simulink model "sm_car"  (R2025a)
settings: Solver=ode23t  StartTime=0.0  StopTime=400  MaxStep=0.4  RelTol=1e-3  AbsTol=1e-3  EnableMultiTasking=on
PreLoadFcn:
  | % Due to usability issue in Repeating Sequence block
  | warning('off','Simulink:Masking:Invalid');
  | 
  | % Eliminate unnecessary warnings in inactive variants
  | % Warnings generated only if you click through inactive variant
  | warning('off','MATLAB:nonExistentField');
  | warning('off','Simulink:Parameters:BlkParamUndefined');
PostLoadFcn:
  | set_param([bdroot '/Vehicle'],'popup_trailer','Off')
  | warning('off','sm:sli:setup:compile:LocalSolverNotSupported')
  | %sm_car_config_maneuver(bdroot,'WOT Braking');
  | sm_car_config_vehicle(bdroot,'false');
  | sm_car_config_logging(bdroot);
InitFcn:
  | sm_car_config_camera;
  | Vehicle = sm_car_vehcfg_checkConfig(Vehicle);
  | sm_car_check_tire_model(bdroot);
StartFcn:
  | tic;
StopFcn:
  | Elapsed_Sim_Time = toc;
  | % disp(['Elapsed Sim Time = ' num2str(Elapsed_Sim_Time)]);
undefined symbols (not defined in the file): Axle1D, AxleIn, Camera, Control, Driver, Free, Init, Maneuver, Pedal, RaceFix, RaceSpin, Scene, ShaftL1, ShaftL2, ShaftR1, ShaftR2, Soft, Stiff, Visual, X, xy_data_car_side, Y, Z
libraries: sm_lib x1546, nesl_utility x528, fl_lib x480, SimscapeFluids_lib x61, sdl_lib x49, simulink x29, ee_lib x7, simulink_extras x6, Linkage_Systems x4, Tire_1x2x x4, AntiRollBar_Systems x2, Linkage_Decoupled x2
(part 57 of 79)

== system sm_car/Vehicle/Vehicle/Chassis/SuspA1/Linkage Decoupled/Steer/Rack Wheel/Driver/None ==
  q : Inport
  Body Sensor Empty : Subsystem  mask{offset_body_sensor=Vehicle.Chassis.Body.sCG.Value}
      mask prompts: offset_body_sensor "Sensor Frame Offset [x y z] (m)"
  Reference Frame : sm_lib/Frames and Transforms/Reference Frame
  Reference Frame1 : sm_lib/Frames and Transforms/Reference Frame
  Reference Frame2 : sm_lib/Frames and Transforms/Reference Frame
  Terminator : Terminator
  HandR : PMIOPort  Side=Right
  HandL : PMIOPort  Port=2  Side=Right
  Ref : PMIOPort  Port=3  Side=Left
  m : Outport  VectorParamsAs1DForOutWhenUnconnected=off
  wires:
  Body Sensor Empty/1(Body) -> m/1
  q/1 -> Terminator/1
  connections:
  Ref/RConn1 -- Reference Frame2/RConn1
  HandL/RConn1 -- Body Sensor Empty/LConn1 -- Reference Frame/RConn1
  Reference Frame1/RConn1 -- HandR/RConn1

== system sm_car/Vehicle/Vehicle/Chassis/SuspA1/Linkage Decoupled/Steer/Rack Wheel/Rack/Transform Suspension Mount ==
  Transform HP Rack : sm_lib/Frames and Transforms/Rigid Transform  RotationMethod=None  FollAlignAxisA=+X  BaseAlignAxisA=+Y  FollAlignAxisB=+Y  BaseAlignAxisB=+Z  RotationStandardAxis=+Z  RotationAngle=0.0  RotationAngleUnits=deg  RotationArbitraryAxis=[0 0 1]  RotationSequenceAxes=FollowerAxes  RotationSequence=XYX  RotationSequenceAngles=[0 0 0]  RotationSequenceAnglesUnits=deg  RotationMatrix=[1 0 0; 0 1 0; 0 0 1]  Quaternion=[1 0 0 0]  TranslationMethod=Cartesian  TranslationCartesianOffset=hp_mt_rack  TranslationCartesianOffsetUnits=m  TranslationStandardAxis=+Z  TranslationStandardOffset=0  TranslationStandardOffsetUnits=m  TranslationROffset=0  TranslationROffsetUnits=m  TranslationThetaOffset=0  TranslationThetaOffsetUnits=deg  TranslationZOffset=0  TranslationZOffsetUnits=m
  Transform Rack Axis : sm_lib/Frames and Transforms/Rigid Transform  RotationMethod=AlignedAxes  FollAlignAxisA=+Y  BaseAlignAxisA=-Z  FollAlignAxisB=+X  BaseAlignAxisB=+X  RotationStandardAxis=+Z  RotationAngle=0  RotationAngleUnits=deg  RotationArbitraryAxis=[0 0 1]  RotationSequenceAxes=FollowerAxes  RotationSequence=XYX  RotationSequenceAngles=[0 0 0]  RotationSequenceAnglesUnits=deg  RotationMatrix=[0 0 -1;0 1 0;1 0 0]  Quaternion=[1 0 0 0]  TranslationMethod=None  TranslationCartesianOffset=[0 0 0]  TranslationCartesianOffsetUnits=m  TranslationStandardAxis=+Z  TranslationStandardOffset=0  TranslationStandardOffsetUnits=m  TranslationROffset=0  TranslationROffsetUnits=m  TranslationThetaOffset=0  TranslationThetaOffsetUnits=deg  TranslationZOffset=0  TranslationZOffsetUnits=m
  B : PMIOPort  Side=Left
  F : PMIOPort  Port=2  Side=Right
  connections:
  Transform Rack Axis/LConn1 -- Transform HP Rack/RConn1
  Transform HP Rack/LConn1 -- B/RConn1
  Transform Rack Axis/RConn1 -- F/RConn1

== system sm_car/Vehicle/Vehicle/Chassis/SuspA1/Linkage Decoupled/Steer/Rack Wheel/Wheel/FSAE ==
  Solid : sm_lib/Body Elements/File Solid  ExtGeomFileName=FSAE_steering_wheel.STEP  UnitType=FromFile  ExtGeomFileUnits=m  StepReaderType=HEX  ExportConvexHullGeometry=off  InertiaType=PointMass  BasedOnType=Density  Density=1000  DensityUnits=kg/m^3  Mass=0  MassUnits=kg  CenterOfMass=[0 0 0]  CenterOfMassUnits=mm  MomentsOfInertia=[1 1 1]  MomentsOfInertiaUnits=kg*mm^2  ProductsOfInertia=[0 0 0]  ProductsOfInertiaUnits=kg*mm^2  GraphicType=FromGeometry  MarkerShape=Sphere  MarkerSize=10  GraphicVisPropType=SimpleVisualProperties  GraphicDiffuseColor=[0.898039215686275 0.917647058823529 0.929411764705882]  GraphicOpacity=1  GraphicSpecularColor=[0.5 0.5 0.5 1.0]  GraphicAmbientColor=[0.15 0.15 0.15 1.0]  GraphicEmissiveColor=[0.0 0.0 0.0 1.0]  GraphicShininess=75  DoExposeReferenceFrame=on  SerializedFrames=<Frames/>
  Transform HandL : sm_lib/Frames and Transforms/Rigid Transform  RotationMethod=AlignedAxes  FollAlignAxisA=+Z  BaseAlignAxisA=-Y  FollAlignAxisB=+X  BaseAlignAxisB=-Z  RotationStandardAxis=+Z  RotationAngle=0  RotationAngleUnits=rad  RotationArbitraryAxis=[0 0 0]  RotationSequenceAxes=FollowerAxes  RotationSequence=XYX  RotationSequenceAngles=[0 0 0]  RotationSequenceAnglesUnits=deg  RotationMatrix=[1 0 0; 0 1 0; 0 0 1]  Quaternion=[1 0 0 0]  TranslationMethod=Cartesian  TranslationCartesianOffset=[-20 130 -10]  TranslationCartesianOffsetUnits=mm  TranslationStandardAxis=+Z  TranslationStandardOffset=0  TranslationStandardOffsetUnits=mm  TranslationROffset=0  TranslationROffsetUnits=m  TranslationThetaOffset=0  TranslationThetaOffsetUnits=deg  TranslationZOffset=0  TranslationZOffsetUnits=m
  Transform HandL Pitch : sm_lib/Frames and Transforms/Rigid Transform  RotationMethod=StandardAxis  FollAlignAxisA=+X  BaseAlignAxisA=+Y  FollAlignAxisB=+Y  BaseAlignAxisB=+Z  RotationStandardAxis=+Z  RotationAngle=20  RotationAngleUnits=deg  RotationArbitraryAxis=[0 0 1]  RotationSequenceAxes=FollowerAxes  RotationSequence=XYX  RotationSequenceAngles=[0 0 0]  RotationSequenceAnglesUnits=deg  RotationMatrix=[1 0 0; 0 1 0; 0 0 1]  Quaternion=[1 0 0 0]  TranslationMethod=None  TranslationCartesianOffset=[0 0 0]  TranslationCartesianOffsetUnits=m  TranslationStandardAxis=+Z  TranslationStandardOffset=0  TranslationStandardOffsetUnits=m  TranslationROffset=0  TranslationROffsetUnits=m  TranslationThetaOffset=0  TranslationThetaOffsetUnits=deg  TranslationZOffset=0  TranslationZOffsetUnits=m
  Transform HandR : sm_lib/Frames and Transforms/Rigid Transform  RotationMethod=AlignedAxes  FollAlignAxisA=+Z  BaseAlignAxisA=-Y  FollAlignAxisB=+X  BaseAlignAxisB=-Z  RotationStandardAxis=+Z  RotationAngle=0  RotationAngleUnits=rad  RotationArbitraryAxis=[0 0 0]  RotationSequenceAxes=FollowerAxes  RotationSequence=XYX  RotationSequenceAngles=[0 0 0]  RotationSequenceAnglesUnits=deg  RotationMatrix=[1 0 0; 0 1 0; 0 0 1]  Quaternion=[1 0 0 0]  TranslationMethod=Cartesian  TranslationCartesianOffset=[-20 -130 -10]  TranslationCartesianOffsetUnits=mm  TranslationStandardAxis=+Z  TranslationStandardOffset=0  TranslationStandardOffsetUnits=mm  TranslationROffset=0  TranslationROffsetUnits=m  TranslationThetaOffset=0  TranslationThetaOffsetUnits=deg  TranslationZOffset=0  TranslationZOffsetUnits=m
  Transform HandR Pitch : sm_lib/Frames and Transforms/Rigid Transform  RotationMethod=StandardAxis  FollAlignAxisA=+X  BaseAlignAxisA=+Y  FollAlignAxisB=+Y  BaseAlignAxisB=+Z  RotationStandardAxis=+Z  RotationAngle=20  RotationAngleUnits=deg  RotationArbitraryAxis=[0 0 1]  RotationSequenceAxes=FollowerAxes  RotationSequence=XYX  RotationSequenceAngles=[0 0 0]  RotationSequenceAnglesUnits=deg  RotationMatrix=[1 0 0; 0 1 0; 0 0 1]  Quaternion=[1 0 0 0]  TranslationMethod=None  TranslationCartesianOffset=[0 0 0]  TranslationCartesianOffsetUnits=m  TranslationStandardAxis=+Z  TranslationStandardOffset=0  TranslationStandardOffsetUnits=m  TranslationROffset=0  TranslationROffsetUnits=m  TranslationThetaOffset=0  TranslationThetaOffsetUnits=deg  TranslationZOffset=0  TranslationZOffsetUnits=m
  Transform Steer Axis : Subsystem
  "SteerAxis  " : PMIOPort  Side=Left
  HandR : PMIOPort  Port=2  Side=Right
  HandL : PMIOPort  Port=3  Side=Right
  connections:
  Transform HandR Pitch/RConn1 -- HandR/RConn1
  Transform HandL Pitch/LConn1 -- Transform HandL/RConn1
  Solid/RConn1 -- Transform Steer Axis/RConn1
  HandL/RConn1 -- Transform HandL Pitch/RConn1
  Transform HandR/RConn1 -- Transform HandR Pitch/LConn1
  Transform Steer Axis/LConn1 -- Transform HandL/LConn1 -- Transform HandR/LConn1 -- "SteerAxis  "/RConn1

== system sm_car/Vehicle/Vehicle/Chassis/SuspA1/Linkage Decoupled/Steer/Rack Wheel/Wheel/Sedan ==
  Reference Frame : sm_lib/Frames and Transforms/Reference Frame
  Steering : Subsystem
  Transform Align HandL : sm_lib/Frames and Transforms/Rigid Transform  RotationMethod=None  FollAlignAxisA=+X  BaseAlignAxisA=+Y  FollAlignAxisB=+Y  BaseAlignAxisB=+Z  RotationStandardAxis=+Z  RotationAngle=0  RotationAngleUnits=deg  RotationArbitraryAxis=[0 0 1]  RotationSequenceAxes=FollowerAxes  RotationSequence=XYX  RotationSequenceAngles=[0 0 0]  RotationSequenceAnglesUnits=deg  RotationMatrix=[1 0 0; 0 1 0; 0 0 1]  Quaternion=[1 0 0 0]  TranslationMethod=StandardAxis  TranslationCartesianOffset=[0 0 0]  TranslationCartesianOffsetUnits=m  TranslationStandardAxis=+Z  TranslationStandardOffset=0.01  TranslationStandardOffsetUnits=m  TranslationROffset=0  TranslationROffsetUnits=m  TranslationThetaOffset=0  TranslationThetaOffsetUnits=deg  TranslationZOffset=0  TranslationZOffsetUnits=m
  Transform HandL : sm_lib/Frames and Transforms/Rigid Transform  RotationMethod=ArbitraryAxis  FollAlignAxisA=+X  BaseAlignAxisA=+Y  FollAlignAxisB=+Y  BaseAlignAxisB=+Z  RotationStandardAxis=+Z  RotationAngle=0  RotationAngleUnits=rad  RotationArbitraryAxis=[0 0 0]  RotationSequenceAxes=FollowerAxes  RotationSequence=XYX  RotationSequenceAngles=[0 0 0]  RotationSequenceAnglesUnits=deg  RotationMatrix=[1 0 0; 0 1 0; 0 0 1]  Quaternion=[1 0 0 0]  TranslationMethod=Cartesian  TranslationCartesianOffset=[75.3002166748051 139.529690146446 17.4556095153098]  TranslationCartesianOffsetUnits=mm  TranslationStandardAxis=+Z  TranslationStandardOffset=0  TranslationStandardOffsetUnits=mm  TranslationROffset=0  TranslationROffsetUnits=m  TranslationThetaOffset=0  TranslationThetaOffsetUnits=deg  TranslationZOffset=0  TranslationZOffsetUnits=m
  Transform Steer Ctr : sm_lib/Frames and Transforms/Rigid Transform  RotationMethod=RotationSequence  FollAlignAxisA=+X  BaseAlignAxisA=+Y  FollAlignAxisB=+Y  BaseAlignAxisB=+Z  RotationStandardAxis=+Z  RotationAngle=0  RotationAngleUnits=deg  RotationArbitraryAxis=[0 0 1]  RotationSequenceAxes=FollowerAxes  RotationSequence=YXZ  RotationSequenceAngles=[-90 -20.218116663649042 90]  RotationSequenceAnglesUnits=deg  RotationMatrix=[1 0 0; 0 1 0; 0 0 1]  Quaternion=[1 0 0 0]  TranslationMethod=Cartesian  TranslationCartesianOffset=[0.072679731994867 0.197345148772001 0]  TranslationCartesianOffsetUnits=m  TranslationStandardAxis=+Z  TranslationStandardOffset=0  TranslationStandardOffsetUnits=m  TranslationROffset=0  TranslationROffsetUnits=m  TranslationThetaOffset=0  TranslationThetaOffsetUnits=deg  TranslationZOffset=0  TranslationZOffsetUnits=m
  Transform HandR : sm_lib/Frames and Transforms/Rigid Transform  RotationMethod=ArbitraryAxis  FollAlignAxisA=+X  BaseAlignAxisA=+Y  FollAlignAxisB=+Y  BaseAlignAxisB=+Z  RotationStandardAxis=+Z  RotationAngle=0  RotationAngleUnits=rad  RotationArbitraryAxis=[0 0 0]  RotationSequenceAxes=FollowerAxes  RotationSequence=XYX  RotationSequenceAngles=[0 0 0]  RotationSequenceAnglesUnits=deg  RotationMatrix=[1 0 0; 0 1 0; 0 0 1]  Quaternion=[1 0 0 0]  TranslationMethod=Cartesian  TranslationCartesianOffset=[75.3002166748047 139.529690146446 404.207736253739]  TranslationCartesianOffsetUnits=mm  TranslationStandardAxis=+Z  TranslationStandardOffset=0  TranslationStandardOffsetUnits=mm  TranslationROffset=0  TranslationROffsetUnits=m  TranslationThetaOffset=0  TranslationThetaOffsetUnits=deg  TranslationZOffset=0  TranslationZOffsetUnits=m
  SteerAxis : PMIOPort  Side=Left
  HandR : PMIOPort  Port=2  Side=Right
  HandL : PMIOPort  Port=3  Side=Right
  connections:
  SteerAxis/RConn1 -- Transform Steer Ctr/RConn1
  Transform HandL/RConn1 -- Transform Align HandL/LConn1
  Steering/LConn1 -- Transform Steer Ctr/LConn1
  Transform Align HandL/RConn1 -- HandL/RConn1
  Transform HandR/RConn1 -- HandR/RConn1
  Transform HandR/LConn1 -- Steering/RConn1 -- Transform HandL/LConn1
  Steering/LConn2 -- Reference Frame/RConn1

== system sm_car/Vehicle/Vehicle/Chassis/SuspA1/Linkage Decoupled/Steer/Rack Wheel ByWire/Driver/Human ==
  q : Inport
  Arm L : Subsystem
  Arm R : Subsystem
  Body Sensor : Subsystem  mask{offset_body_sensor=Vehicle.Chassis.Body.sCG.Value}
      mask prompts: offset_body_sensor "Sensor Frame Offset [x y z] (m)"
  Gain : Gain  Gain=-1
  Head : Subsystem
  Leg L : Subsystem
  Leg R : Subsystem
  Pelvis : Subsystem
  Revolute Neck : sm_lib/Joints/Revolute Joint  JointMode=Normal  CompositeWrenchDir=FollowerOnBase  CompositeWrenchFrame=BaseFrame  SenseConstraintForce=off  SenseConstraintTorque=off  SenseTotalForce=off  SenseTotalTorque=off  PositionTargetSpecify=on  PositionTargetPriority=Low  PositionTargetValue=0  PositionTargetValueUnits=deg  VelocityTargetSpecify=off  VelocityTargetPriority=High  VelocityTargetValue=0  VelocityTargetValueUnits=deg/s  EquilibriumPosition=0  EquilibriumPositionUnits=rad  SpringStiffness=0  SpringStiffnessUnits=N*m/rad  DampingCoefficient=0  DampingCoefficientUnits=N*m/(rad/s)  LowerLimitSpecify=off  LowerLimitBound=-90  LowerLimitBoundUnits=deg  LowerLimitStiffness=1e4  LowerLimitStiffnessUnits=N*m/deg  LowerLimitDamping=10  LowerLimitDampingUnits=N*m/(deg/s)  LowerLimitTransitionRegionWidth=0.1  LowerLimitTransitionRegionWidthUnits=deg  UpperLimitSpecify=off  UpperLimitBound=90  UpperLimitBoundUnits=deg  UpperLimitStiffness=1e4  UpperLimitStiffnessUnits=N*m/deg  UpperLimitDamping=10  UpperLimitDampingUnits=N*m/(deg/s)  UpperLimitTransitionRegionWidth=0.1  UpperLimitTransitionRegionWidthUnits=deg  TorqueActuationMode=ComputedTorque  MotionActuationMode=InputMotion  SensePosition=off  SenseVelocity=off  SenseAcceleration=off  SenseTorqueForce=off  SenseLowerLimitTorqueForce=off  SenseUpperLimitTorqueForce=off
  Simulink-PS Converter : nesl_utility/Simulink-PS Converter  PhysicalDomain=network_engine_domain  SubClassName=ps_input  LeftPortType=input  RightPortType=output  PseudoPeriodic=off  Frequencies=[]  NoiseDistribution=none  NoiseParameters=[]  Unit=rad  AffineConversion=off  FilteringAndDerivatives=filter  SimscapeFilterOrder=2  InputFilterTimeConstant=0.1  UdotUserProvided=0
  Torso : Subsystem
  Transform FA to Driver : sm_lib/Frames and Transforms/Rigid Transform  RotationMethod=RotationSequence  FollAlignAxisA=+X  BaseAlignAxisA=+Y  FollAlignAxisB=+Y  BaseAlignAxisB=+Z  RotationStandardAxis=+Z  RotationAngle=0.0  RotationAngleUnits=deg  RotationArbitraryAxis=[0 0 1]  RotationSequenceAxes=FollowerAxes  RotationSequence=ZYX  RotationSequenceAngles=[rpy_human(3) rpy_human(2) rpy_human(1)]  RotationSequenceAnglesUnits=deg  RotationMatrix=[1 0 0; 0 1 0; 0 0 1]  Quaternion=[1 0 0 0]  TranslationMethod=Cartesian  TranslationCartesianOffset=hp_human  TranslationCartesianOffsetUnits=m  TranslationStandardAxis=+Z  TranslationStandardOffset=0  TranslationStandardOffsetUnits=m  TranslationROffset=0  TranslationROffsetUnits=m  TranslationThetaOffset=0  TranslationThetaOffsetUnits=deg  TranslationZOffset=0  TranslationZOffsetUnits=m
  Transform Seat Angle : sm_lib/Frames and Transforms/Rigid Transform  RotationMethod=StandardAxis  FollAlignAxisA=+X  BaseAlignAxisA=+Y  FollAlignAxisB=+Y  BaseAlignAxisB=+Z  RotationStandardAxis=+Y  RotationAngle=143.2261743756  RotationAngleUnits=deg  RotationArbitraryAxis=[0 0 1]  RotationSequenceAxes=FollowerAxes  RotationSequence=XYX  RotationSequenceAngles=[0 0 0]  RotationSequenceAnglesUnits=deg  RotationMatrix=[1 0 0; 0 1 0; 0 0 1]  Quaternion=[1 0 0 0]  TranslationMethod=None  TranslationCartesianOffset=[0 0 0]  TranslationCartesianOffsetUnits=m  TranslationStandardAxis=+Z  TranslationStandardOffset=0  TranslationStandardOffsetUnits=m  TranslationROffset=0  TranslationROffsetUnits=m  TranslationThetaOffset=0  TranslationThetaOffsetUnits=deg  TranslationZOffset=0  TranslationZOffsetUnits=m
  Twist : Subsystem
  HandR : PMIOPort  Side=Right
  HandL : PMIOPort  Port=2  Side=Right
  Ref : PMIOPort  Port=3  Side=Left
  m : Outport  VectorParamsAs1DForOutWhenUnconnected=off
  wires:
  Body Sensor/1(Body) -> m/1
  Gain/1 -> Simulink-PS Converter/1
  q/1 -> Gain/1
  connections:
  Body Sensor/LConn1 -- Head/RConn1
  Transform Seat Angle/RConn1 -- Transform FA to Driver/RConn1
  Head/LConn1 -- Revolute Neck/RConn1
  Revolute Neck/LConn1 -- Torso/RConn2
  Pelvis/RConn2 -- Leg R/LConn1
  Leg L/LConn1 -- Pelvis/RConn1
  Arm R/RConn1 -- HandR/RConn1
  Torso/RConn3 -- Arm R/LConn1
  Arm L/LConn1 -- Torso/RConn1
  Arm L/RConn1 -- HandL/RConn1
  Twist/RConn1 -- Torso/LConn1
  Pelvis/LConn1 -- Twist/LConn1 -- Transform Seat Angle/LConn1
  Transform FA to Driver/LConn1 -- Ref/RConn1
  Simulink-PS Converter/RConn1 -- Revolute Neck/LConn2

== system sm_car/Vehicle/Vehicle/Chassis/SuspA1/Linkage Decoupled/Steer/Rack Wheel ByWire/Driver/None ==
  q : Inport
  Body Sensor Empty : Subsystem  mask{offset_body_sensor=Vehicle.Chassis.Body.sCG.Value}
      mask prompts: offset_body_sensor "Sensor Frame Offset [x y z] (m)"
  Reference Frame : sm_lib/Frames and Transforms/Reference Frame
  Reference Frame1 : sm_lib/Frames and Transforms/Reference Frame
  Reference Frame2 : sm_lib/Frames and Transforms/Reference Frame
  Terminator : Terminator
  HandR : PMIOPort  Side=Right
  HandL : PMIOPort  Port=2  Side=Right
  Ref : PMIOPort  Port=3  Side=Left
  m : Outport  VectorParamsAs1DForOutWhenUnconnected=off
  wires:
  Body Sensor Empty/1(Body) -> m/1
  q/1 -> Terminator/1
  connections:
  Ref/RConn1 -- Reference Frame2/RConn1
  HandL/RConn1 -- Body Sensor Empty/LConn1 -- Reference Frame/RConn1
  Reference Frame1/RConn1 -- HandR/RConn1

== system sm_car/Vehicle/Vehicle/Chassis/SuspA1/Linkage Decoupled/Steer/Rack Wheel ByWire/Motors/Control ==
  Meas : Inport
  Cmd : Inport  Port=2
  Abs : Abs  ZeroCross=off  SaturateOnIntegerOverflow=off
  Derivative : TransferFcn  Numerator=[1 0]  Denominator=[tFilt_deriv 1]
  Filter xRack : simulink_extras/Additional Linear/Transfer Fcn (with initial states)  N=[1]  D=[tFilt_xRack 1]  X0=0
  Integrator : Integrator
  Kd : Gain  Gain=Kd
  Ki : Gain  Gain=Ki
  Kp : Lookup_n-D  NumberOfTableDimensions=1  BreakpointsForDimension1=Kp_breakpoints  Table=Kp_values  InternalRulePriority=Speed  RndMeth=Simplest
  Product : Product
  Product1 : Product
  Steer Torque Factor : Constant  Value=nTrqSteer
  Sum : Sum  Inputs=+-|
  Sum1 : Sum  Inputs=+++
  trqRack : Outport
  trqSteer : Outport  Port=2
  wires:
  Cmd/1 -> Sum/1, Abs/1
  Meas/1 -> Filter xRack/1
  Sum/1 -> Ki/1, Product/2, Kd/1
  Integrator/1 -> Sum1/2
  Ki/1 -> Integrator/1
  Product/1 -> Sum1/1
  Kd/1 -> Derivative/1
  Derivative/1 -> Sum1/3
  Filter xRack/1 -> Sum/2
  Kp/1 -> Product/1
  Abs/1 -> Kp/1
  Steer Torque Factor/1 -> Product1/1
  Product1/1 -> trqSteer/1
  Sum1/1 -> Product1/2, trqRack/1

== system sm_car/Vehicle/Vehicle/Chassis/SuspA1/Linkage Decoupled/Steer/Rack Wheel ByWire/Rack/Transform Suspension Mount ==
  Transform HP Rack : sm_lib/Frames and Transforms/Rigid Transform  RotationMethod=None  FollAlignAxisA=+X  BaseAlignAxisA=+Y  FollAlignAxisB=+Y  BaseAlignAxisB=+Z  RotationStandardAxis=+Z  RotationAngle=0.0  RotationAngleUnits=deg  RotationArbitraryAxis=[0 0 1]  RotationSequenceAxes=FollowerAxes  RotationSequence=XYX  RotationSequenceAngles=[0 0 0]  RotationSequenceAnglesUnits=deg  RotationMatrix=[1 0 0; 0 1 0; 0 0 1]  Quaternion=[1 0 0 0]  TranslationMethod=Cartesian  TranslationCartesianOffset=hp_mt_rack  TranslationCartesianOffsetUnits=m  TranslationStandardAxis=+Z  TranslationStandardOffset=0  TranslationStandardOffsetUnits=m  TranslationROffset=0  TranslationROffsetUnits=m  TranslationThetaOffset=0  TranslationThetaOffsetUnits=deg  TranslationZOffset=0  TranslationZOffsetUnits=m
  Transform Rack Axis : sm_lib/Frames and Transforms/Rigid Transform  RotationMethod=AlignedAxes  FollAlignAxisA=+Y  BaseAlignAxisA=-Z  FollAlignAxisB=+X  BaseAlignAxisB=+X  RotationStandardAxis=+Z  RotationAngle=0  RotationAngleUnits=deg  RotationArbitraryAxis=[0 0 1]  RotationSequenceAxes=FollowerAxes  RotationSequence=XYX  RotationSequenceAngles=[0 0 0]  RotationSequenceAnglesUnits=deg  RotationMatrix=[0 0 -1;0 1 0;1 0 0]  Quaternion=[1 0 0 0]  TranslationMethod=None  TranslationCartesianOffset=[0 0 0]  TranslationCartesianOffsetUnits=m  TranslationStandardAxis=+Z  TranslationStandardOffset=0  TranslationStandardOffsetUnits=m  TranslationROffset=0  TranslationROffsetUnits=m  TranslationThetaOffset=0  TranslationThetaOffsetUnits=deg  TranslationZOffset=0  TranslationZOffsetUnits=m
  B : PMIOPort  Side=Left
  F : PMIOPort  Port=2  Side=Right
  connections:
  Transform Rack Axis/LConn1 -- Transform HP Rack/RConn1
  Transform HP Rack/LConn1 -- B/RConn1
  Transform Rack Axis/RConn1 -- F/RConn1

== system sm_car/Vehicle/Vehicle/Chassis/SuspA1/Linkage Decoupled/Steer/Rack Wheel ByWire/Wheel/FSAE ==
  Solid : sm_lib/Body Elements/File Solid  ExtGeomFileName=FSAE_steering_wheel.STEP  UnitType=FromFile  ExtGeomFileUnits=m  StepReaderType=HEX  ExportConvexHullGeometry=off  InertiaType=PointMass  BasedOnType=Density  Density=1000  DensityUnits=kg/m^3  Mass=0  MassUnits=kg  CenterOfMass=[0 0 0]  CenterOfMassUnits=mm  MomentsOfInertia=[1 1 1]  MomentsOfInertiaUnits=kg*mm^2  ProductsOfInertia=[0 0 0]  ProductsOfInertiaUnits=kg*mm^2  GraphicType=FromGeometry  MarkerShape=Sphere  MarkerSize=10  GraphicVisPropType=SimpleVisualProperties  GraphicDiffuseColor=[0.898039215686275 0.917647058823529 0.929411764705882]  GraphicOpacity=1  GraphicSpecularColor=[0.5 0.5 0.5 1.0]  GraphicAmbientColor=[0.15 0.15 0.15 1.0]  GraphicEmissiveColor=[0.0 0.0 0.0 1.0]  GraphicShininess=75  DoExposeReferenceFrame=on  SerializedFrames=<Frames/>
  Transform HandL : sm_lib/Frames and Transforms/Rigid Transform  RotationMethod=AlignedAxes  FollAlignAxisA=+Z  BaseAlignAxisA=-Y  FollAlignAxisB=+X  BaseAlignAxisB=-Z  RotationStandardAxis=+Z  RotationAngle=0  RotationAngleUnits=rad  RotationArbitraryAxis=[0 0 0]  RotationSequenceAxes=FollowerAxes  RotationSequence=XYX  RotationSequenceAngles=[0 0 0]  RotationSequenceAnglesUnits=deg  RotationMatrix=[1 0 0; 0 1 0; 0 0 1]  Quaternion=[1 0 0 0]  TranslationMethod=Cartesian  TranslationCartesianOffset=[-20 130 -10]  TranslationCartesianOffsetUnits=mm  TranslationStandardAxis=+Z  TranslationStandardOffset=0  TranslationStandardOffsetUnits=mm  TranslationROffset=0  TranslationROffsetUnits=m  TranslationThetaOffset=0  TranslationThetaOffsetUnits=deg  TranslationZOffset=0  TranslationZOffsetUnits=m
  Transform HandL Pitch : sm_lib/Frames and Transforms/Rigid Transform  RotationMethod=StandardAxis  FollAlignAxisA=+X  BaseAlignAxisA=+Y  FollAlignAxisB=+Y  BaseAlignAxisB=+Z  RotationStandardAxis=+Z  RotationAngle=20  RotationAngleUnits=deg  RotationArbitraryAxis=[0 0 1]  RotationSequenceAxes=FollowerAxes  RotationSequence=XYX  RotationSequenceAngles=[0 0 0]  RotationSequenceAnglesUnits=deg  RotationMatrix=[1 0 0; 0 1 0; 0 0 1]  Quaternion=[1 0 0 0]  TranslationMethod=None  TranslationCartesianOffset=[0 0 0]  TranslationCartesianOffsetUnits=m  TranslationStandardAxis=+Z  TranslationStandardOffset=0  TranslationStandardOffsetUnits=m  TranslationROffset=0  TranslationROffsetUnits=m  TranslationThetaOffset=0  TranslationThetaOffsetUnits=deg  TranslationZOffset=0  TranslationZOffsetUnits=m
  Transform HandR : sm_lib/Frames and Transforms/Rigid Transform  RotationMethod=AlignedAxes  FollAlignAxisA=+Z  BaseAlignAxisA=-Y  FollAlignAxisB=+X  BaseAlignAxisB=-Z  RotationStandardAxis=+Z  RotationAngle=0  RotationAngleUnits=rad  RotationArbitraryAxis=[0 0 0]  RotationSequenceAxes=FollowerAxes  RotationSequence=XYX  RotationSequenceAngles=[0 0 0]  RotationSequenceAnglesUnits=deg  RotationMatrix=[1 0 0; 0 1 0; 0 0 1]  Quaternion=[1 0 0 0]  TranslationMethod=Cartesian  TranslationCartesianOffset=[-20 -130 -10]  TranslationCartesianOffsetUnits=mm  TranslationStandardAxis=+Z  TranslationStandardOffset=0  TranslationStandardOffsetUnits=mm  TranslationROffset=0  TranslationROffsetUnits=m  TranslationThetaOffset=0  TranslationThetaOffsetUnits=deg  TranslationZOffset=0  TranslationZOffsetUnits=m
  Transform HandR Pitch : sm_lib/Frames and Transforms/Rigid Transform  RotationMethod=StandardAxis  FollAlignAxisA=+X  BaseAlignAxisA=+Y  FollAlignAxisB=+Y  BaseAlignAxisB=+Z  RotationStandardAxis=+Z  RotationAngle=20  RotationAngleUnits=deg  RotationArbitraryAxis=[0 0 1]  RotationSequenceAxes=FollowerAxes  RotationSequence=XYX  RotationSequenceAngles=[0 0 0]  RotationSequenceAnglesUnits=deg  RotationMatrix=[1 0 0; 0 1 0; 0 0 1]  Quaternion=[1 0 0 0]  TranslationMethod=None  TranslationCartesianOffset=[0 0 0]  TranslationCartesianOffsetUnits=m  TranslationStandardAxis=+Z  TranslationStandardOffset=0  TranslationStandardOffsetUnits=m  TranslationROffset=0  TranslationROffsetUnits=m  TranslationThetaOffset=0  TranslationThetaOffsetUnits=deg  TranslationZOffset=0  TranslationZOffsetUnits=m
  Transform Steer Axis : Subsystem
  "SteerAxis  " : PMIOPort  Side=Left
  HandR : PMIOPort  Port=2  Side=Right
  HandL : PMIOPort  Port=3  Side=Right
  connections:
  Transform HandR Pitch/RConn1 -- HandR/RConn1
  Transform HandL Pitch/LConn1 -- Transform HandL/RConn1
  Solid/RConn1 -- Transform Steer Axis/RConn1
  HandL/RConn1 -- Transform HandL Pitch/RConn1
  Transform HandR/RConn1 -- Transform HandR Pitch/LConn1
  Transform Steer Axis/LConn1 -- Transform HandL/LConn1 -- Transform HandR/LConn1 -- "SteerAxis  "/RConn1

== system sm_car/Vehicle/Vehicle/Chassis/SuspA1/Linkage Decoupled/Steer/Rack Wheel ByWire/Wheel/Sedan ==
  Reference Frame : sm_lib/Frames and Transforms/Reference Frame
  Steering : Subsystem
  Transform Align HandL : sm_lib/Frames and Transforms/Rigid Transform  RotationMethod=None  FollAlignAxisA=+X  BaseAlignAxisA=+Y  FollAlignAxisB=+Y  BaseAlignAxisB=+Z  RotationStandardAxis=+Z  RotationAngle=0  RotationAngleUnits=deg  RotationArbitraryAxis=[0 0 1]  RotationSequenceAxes=FollowerAxes  RotationSequence=XYX  RotationSequenceAngles=[0 0 0]  RotationSequenceAnglesUnits=deg  RotationMatrix=[1 0 0; 0 1 0; 0 0 1]  Quaternion=[1 0 0 0]  TranslationMethod=StandardAxis  TranslationCartesianOffset=[0 0 0]  TranslationCartesianOffsetUnits=m  TranslationStandardAxis=+Z  TranslationStandardOffset=0.01  TranslationStandardOffsetUnits=m  TranslationROffset=0  TranslationROffsetUnits=m  TranslationThetaOffset=0  TranslationThetaOffsetUnits=deg  TranslationZOffset=0  TranslationZOffsetUnits=m
  Transform HandL : sm_lib/Frames and Transforms/Rigid Transform  RotationMethod=ArbitraryAxis  FollAlignAxisA=+X  BaseAlignAxisA=+Y  FollAlignAxisB=+Y  BaseAlignAxisB=+Z  RotationStandardAxis=+Z  RotationAngle=0  RotationAngleUnits=rad  RotationArbitraryAxis=[0 0 0]  RotationSequenceAxes=FollowerAxes  RotationSequence=XYX  RotationSequenceAngles=[0 0 0]  RotationSequenceAnglesUnits=deg  RotationMatrix=[1 0 0; 0 1 0; 0 0 1]  Quaternion=[1 0 0 0]  TranslationMethod=Cartesian  TranslationCartesianOffset=[75.3002166748051 139.529690146446 17.4556095153098]  TranslationCartesianOffsetUnits=mm  TranslationStandardAxis=+Z  TranslationStandardOffset=0  TranslationStandardOffsetUnits=mm  TranslationROffset=0  TranslationROffsetUnits=m  TranslationThetaOffset=0  TranslationThetaOffsetUnits=deg  TranslationZOffset=0  TranslationZOffsetUnits=m
  Transform Steer Ctr : sm_lib/Frames and Transforms/Rigid Transform  RotationMethod=RotationSequence  FollAlignAxisA=+X  BaseAlignAxisA=+Y  FollAlignAxisB=+Y  BaseAlignAxisB=+Z  RotationStandardAxis=+Z  RotationAngle=0  RotationAngleUnits=deg  RotationArbitraryAxis=[0 0 1]  RotationSequenceAxes=FollowerAxes  RotationSequence=YXZ  RotationSequenceAngles=[-90 -20.218116663649042 90]  RotationSequenceAnglesUnits=deg  RotationMatrix=[1 0 0; 0 1 0; 0 0 1]  Quaternion=[1 0 0 0]  TranslationMethod=Cartesian  TranslationCartesianOffset=[0.072679731994867 0.197345148772001 0]  TranslationCartesianOffsetUnits=m  TranslationStandardAxis=+Z  TranslationStandardOffset=0  TranslationStandardOffsetUnits=m  TranslationROffset=0  TranslationROffsetUnits=m  TranslationThetaOffset=0  TranslationThetaOffsetUnits=deg  TranslationZOffset=0  TranslationZOffsetUnits=m
  Transform HandR : sm_lib/Frames and Transforms/Rigid Transform  RotationMethod=ArbitraryAxis  FollAlignAxisA=+X  BaseAlignAxisA=+Y  FollAlignAxisB=+Y  BaseAlignAxisB=+Z  RotationStandardAxis=+Z  RotationAngle=0  RotationAngleUnits=rad  RotationArbitraryAxis=[0 0 0]  RotationSequenceAxes=FollowerAxes  RotationSequence=XYX  RotationSequenceAngles=[0 0 0]  RotationSequenceAnglesUnits=deg  RotationMatrix=[1 0 0; 0 1 0; 0 0 1]  Quaternion=[1 0 0 0]  TranslationMethod=Cartesian  TranslationCartesianOffset=[75.3002166748047 139.529690146446 404.207736253739]  TranslationCartesianOffsetUnits=mm  TranslationStandardAxis=+Z  TranslationStandardOffset=0  TranslationStandardOffsetUnits=mm  TranslationROffset=0  TranslationROffsetUnits=m  TranslationThetaOffset=0  TranslationThetaOffsetUnits=deg  TranslationZOffset=0  TranslationZOffsetUnits=m
  SteerAxis : PMIOPort  Side=Left
  HandR : PMIOPort  Port=2  Side=Right
  HandL : PMIOPort  Port=3  Side=Right
  connections:
  SteerAxis/RConn1 -- Transform Steer Ctr/RConn1
  Transform HandL/RConn1 -- Transform Align HandL/LConn1
  Steering/LConn1 -- Transform Steer Ctr/LConn1
  Transform Align HandL/RConn1 -- HandL/RConn1
  Transform HandR/RConn1 -- HandR/RConn1
  Transform HandR/LConn1 -- Steering/RConn1 -- Transform HandL/LConn1
  Steering/LConn2 -- Reference Frame/RConn1

== system sm_car/Vehicle/Vehicle/Chassis/SuspA1/Linkage Decoupled/Steer/Rack Wheel Indep/Driver/Human ==
  q : Inport
  Arm L : Subsystem
  Arm R : Subsystem
  Body Sensor : Subsystem  mask{offset_body_sensor=Vehicle.Chassis.Body.sCG.Value}
      mask prompts: offset_body_sensor "Sensor Frame Offset [x y z] (m)"
  Gain : Gain  Gain=-1
  Head : Subsystem
  Leg L : Subsystem
  Leg R : Subsystem
  Pelvis : Subsystem
  Revolute Neck : sm_lib/Joints/Revolute Joint  JointMode=Normal  CompositeWrenchDir=FollowerOnBase  CompositeWrenchFrame=BaseFrame  SenseConstraintForce=off  SenseConstraintTorque=off  SenseTotalForce=off  SenseTotalTorque=off  PositionTargetSpecify=on  PositionTargetPriority=Low  PositionTargetValue=0  PositionTargetValueUnits=deg  VelocityTargetSpecify=off  VelocityTargetPriority=High  VelocityTargetValue=0  VelocityTargetValueUnits=deg/s  EquilibriumPosition=0  EquilibriumPositionUnits=rad  SpringStiffness=0  SpringStiffnessUnits=N*m/rad  DampingCoefficient=0  DampingCoefficientUnits=N*m/(rad/s)  LowerLimitSpecify=off  LowerLimitBound=-90  LowerLimitBoundUnits=deg  LowerLimitStiffness=1e4  LowerLimitStiffnessUnits=N*m/deg  LowerLimitDamping=10  LowerLimitDampingUnits=N*m/(deg/s)  LowerLimitTransitionRegionWidth=0.1  LowerLimitTransitionRegionWidthUnits=deg  UpperLimitSpecify=off  UpperLimitBound=90  UpperLimitBoundUnits=deg  UpperLimitStiffness=1e4  UpperLimitStiffnessUnits=N*m/deg  UpperLimitDamping=10  UpperLimitDampingUnits=N*m/(deg/s)  UpperLimitTransitionRegionWidth=0.1  UpperLimitTransitionRegionWidthUnits=deg  TorqueActuationMode=ComputedTorque  MotionActuationMode=InputMotion  SensePosition=off  SenseVelocity=off  SenseAcceleration=off  SenseTorqueForce=off  SenseLowerLimitTorqueForce=off  SenseUpperLimitTorqueForce=off
  Simulink-PS Converter : nesl_utility/Simulink-PS Converter  PhysicalDomain=network_engine_domain  SubClassName=ps_input  LeftPortType=input  RightPortType=output  PseudoPeriodic=off  Frequencies=[]  NoiseDistribution=none  NoiseParameters=[]  Unit=rad  AffineConversion=off  FilteringAndDerivatives=filter  SimscapeFilterOrder=2  InputFilterTimeConstant=0.1  UdotUserProvided=0
  Torso : Subsystem
  Transform FA to Driver : sm_lib/Frames and Transforms/Rigid Transform  RotationMethod=RotationSequence  FollAlignAxisA=+X  BaseAlignAxisA=+Y  FollAlignAxisB=+Y  BaseAlignAxisB=+Z  RotationStandardAxis=+Z  RotationAngle=0.0  RotationAngleUnits=deg  RotationArbitraryAxis=[0 0 1]  RotationSequenceAxes=FollowerAxes  RotationSequence=ZYX  RotationSequenceAngles=[rpy_human(3) rpy_human(2) rpy_human(1)]  RotationSequenceAnglesUnits=deg  RotationMatrix=[1 0 0; 0 1 0; 0 0 1]  Quaternion=[1 0 0 0]  TranslationMethod=Cartesian  TranslationCartesianOffset=hp_human  TranslationCartesianOffsetUnits=m  TranslationStandardAxis=+Z  TranslationStandardOffset=0  TranslationStandardOffsetUnits=m  TranslationROffset=0  TranslationROffsetUnits=m  TranslationThetaOffset=0  TranslationThetaOffsetUnits=deg  TranslationZOffset=0  TranslationZOffsetUnits=m
  Transform Seat Angle : sm_lib/Frames and Transforms/Rigid Transform  RotationMethod=StandardAxis  FollAlignAxisA=+X  BaseAlignAxisA=+Y  FollAlignAxisB=+Y  BaseAlignAxisB=+Z  RotationStandardAxis=+Y  RotationAngle=143.2261743756  RotationAngleUnits=deg  RotationArbitraryAxis=[0 0 1]  RotationSequenceAxes=FollowerAxes  RotationSequence=XYX  RotationSequenceAngles=[0 0 0]  RotationSequenceAnglesUnits=deg  RotationMatrix=[1 0 0; 0 1 0; 0 0 1]  Quaternion=[1 0 0 0]  TranslationMethod=None  TranslationCartesianOffset=[0 0 0]  TranslationCartesianOffsetUnits=m  TranslationStandardAxis=+Z  TranslationStandardOffset=0  TranslationStandardOffsetUnits=m  TranslationROffset=0  TranslationROffsetUnits=m  TranslationThetaOffset=0  TranslationThetaOffsetUnits=deg  TranslationZOffset=0  TranslationZOffsetUnits=m
  Twist : Subsystem
  HandR : PMIOPort  Side=Right
  HandL : PMIOPort  Port=2  Side=Right
  Ref : PMIOPort  Port=3  Side=Left
  m : Outport  VectorParamsAs1DForOutWhenUnconnected=off
  wires:
  Body Sensor/1(Body) -> m/1
  Gain/1 -> Simulink-PS Converter/1
  q/1 -> Gain/1
  connections:
  Body Sensor/LConn1 -- Head/RConn1
  Transform Seat Angle/RConn1 -- Transform FA to Driver/RConn1
  Head/LConn1 -- Revolute Neck/RConn1
  Revolute Neck/LConn1 -- Torso/RConn2
  Pelvis/RConn2 -- Leg R/LConn1
  Leg L/LConn1 -- Pelvis/RConn1
  Arm R/RConn1 -- HandR/RConn1
  Torso/RConn3 -- Arm R/LConn1
  Arm L/LConn1 -- Torso/RConn1
  Arm L/RConn1 -- HandL/RConn1
  Twist/RConn1 -- Torso/LConn1
  Pelvis/LConn1 -- Twist/LConn1 -- Transform Seat Angle/LConn1
  Transform FA to Driver/LConn1 -- Ref/RConn1
  Simulink-PS Converter/RConn1 -- Revolute Neck/LConn2

== system sm_car/Vehicle/Vehicle/Chassis/SuspA1/Linkage Decoupled/Steer/Rack Wheel Indep/Driver/None ==
  q : Inport
  Body Sensor Empty : Subsystem  mask{offset_body_sensor=Vehicle.Chassis.Body.sCG.Value}
      mask prompts: offset_body_sensor "Sensor Frame Offset [x y z] (m)"
  Reference Frame : sm_lib/Frames and Transforms/Reference Frame
  Reference Frame1 : sm_lib/Frames and Transforms/Reference Frame
  Reference Frame2 : sm_lib/Frames and Transforms/Reference Frame
  Terminator : Terminator
  HandR : PMIOPort  Side=Right
  HandL : PMIOPort  Port=2  Side=Right
  Ref : PMIOPort  Port=3  Side=Left
  m : Outport  VectorParamsAs1DForOutWhenUnconnected=off
  wires:
  Body Sensor Empty/1(Body) -> m/1
  q/1 -> Terminator/1
  connections:
  Ref/RConn1 -- Reference Frame2/RConn1
  HandL/RConn1 -- Body Sensor Empty/LConn1 -- Reference Frame/RConn1
  Reference Frame1/RConn1 -- HandR/RConn1

== system sm_car/Vehicle/Vehicle/Chassis/SuspA1/Linkage Decoupled/Steer/Rack Wheel Indep/Rack/Transform Suspension Mount ==
  Transform HP Rack : sm_lib/Frames and Transforms/Rigid Transform  RotationMethod=None  FollAlignAxisA=+X  BaseAlignAxisA=+Y  FollAlignAxisB=+Y  BaseAlignAxisB=+Z  RotationStandardAxis=+Z  RotationAngle=0.0  RotationAngleUnits=deg  RotationArbitraryAxis=[0 0 1]  RotationSequenceAxes=FollowerAxes  RotationSequence=XYX  RotationSequenceAngles=[0 0 0]  RotationSequenceAnglesUnits=deg  RotationMatrix=[1 0 0; 0 1 0; 0 0 1]  Quaternion=[1 0 0 0]  TranslationMethod=Cartesian  TranslationCartesianOffset=hp_mt_rack  TranslationCartesianOffsetUnits=m  TranslationStandardAxis=+Z  TranslationStandardOffset=0  TranslationStandardOffsetUnits=m  TranslationROffset=0  TranslationROffsetUnits=m  TranslationThetaOffset=0  TranslationThetaOffsetUnits=deg  TranslationZOffset=0  TranslationZOffsetUnits=m
  Transform Rack Axis : sm_lib/Frames and Transforms/Rigid Transform  RotationMethod=AlignedAxes  FollAlignAxisA=+Y  BaseAlignAxisA=-Z  FollAlignAxisB=+X  BaseAlignAxisB=+X  RotationStandardAxis=+Z  RotationAngle=0  RotationAngleUnits=deg  RotationArbitraryAxis=[0 0 1]  RotationSequenceAxes=FollowerAxes  RotationSequence=XYX  RotationSequenceAngles=[0 0 0]  RotationSequenceAnglesUnits=deg  RotationMatrix=[0 0 -1;0 1 0;1 0 0]  Quaternion=[1 0 0 0]  TranslationMethod=None  TranslationCartesianOffset=[0 0 0]  TranslationCartesianOffsetUnits=m  TranslationStandardAxis=+Z  TranslationStandardOffset=0  TranslationStandardOffsetUnits=m  TranslationROffset=0  TranslationROffsetUnits=m  TranslationThetaOffset=0  TranslationThetaOffsetUnits=deg  TranslationZOffset=0  TranslationZOffsetUnits=m
  B : PMIOPort  Side=Left
  F : PMIOPort  Port=2  Side=Right
  connections:
  Transform Rack Axis/LConn1 -- Transform HP Rack/RConn1
  Transform HP Rack/LConn1 -- B/RConn1
  Transform Rack Axis/RConn1 -- F/RConn1

== system sm_car/Vehicle/Vehicle/Chassis/SuspA1/Linkage Decoupled/Steer/Rack Wheel Indep/Wheel/FSAE ==
  Solid : sm_lib/Body Elements/File Solid  ExtGeomFileName=FSAE_steering_wheel.STEP  UnitType=FromFile  ExtGeomFileUnits=m  StepReaderType=HEX  ExportConvexHullGeometry=off  InertiaType=PointMass  BasedOnType=Density  Density=1000  DensityUnits=kg/m^3  Mass=0  MassUnits=kg  CenterOfMass=[0 0 0]  CenterOfMassUnits=mm  MomentsOfInertia=[1 1 1]  MomentsOfInertiaUnits=kg*mm^2  ProductsOfInertia=[0 0 0]  ProductsOfInertiaUnits=kg*mm^2  GraphicType=FromGeometry  MarkerShape=Sphere  MarkerSize=10  GraphicVisPropType=SimpleVisualProperties  GraphicDiffuseColor=[0.898039215686275 0.917647058823529 0.929411764705882]  GraphicOpacity=1  GraphicSpecularColor=[0.5 0.5 0.5 1.0]  GraphicAmbientColor=[0.15 0.15 0.15 1.0]  GraphicEmissiveColor=[0.0 0.0 0.0 1.0]  GraphicShininess=75  DoExposeReferenceFrame=on  SerializedFrames=<Frames/>
  Transform HandL : sm_lib/Frames and Transforms/Rigid Transform  RotationMethod=AlignedAxes  FollAlignAxisA=+Z  BaseAlignAxisA=-Y  FollAlignAxisB=+X  BaseAlignAxisB=-Z  RotationStandardAxis=+Z  RotationAngle=0  RotationAngleUnits=rad  RotationArbitraryAxis=[0 0 0]  RotationSequenceAxes=FollowerAxes  RotationSequence=XYX  RotationSequenceAngles=[0 0 0]  RotationSequenceAnglesUnits=deg  RotationMatrix=[1 0 0; 0 1 0; 0 0 1]  Quaternion=[1 0 0 0]  TranslationMethod=Cartesian  TranslationCartesianOffset=[-20 130 -10]  TranslationCartesianOffsetUnits=mm  TranslationStandardAxis=+Z  TranslationStandardOffset=0  TranslationStandardOffsetUnits=mm  TranslationROffset=0  TranslationROffsetUnits=m  TranslationThetaOffset=0  TranslationThetaOffsetUnits=deg  TranslationZOffset=0  TranslationZOffsetUnits=m
  Transform HandL Pitch : sm_lib/Frames and Transforms/Rigid Transform  RotationMethod=StandardAxis  FollAlignAxisA=+X  BaseAlignAxisA=+Y  FollAlignAxisB=+Y  BaseAlignAxisB=+Z  RotationStandardAxis=+Z  RotationAngle=20  RotationAngleUnits=deg  RotationArbitraryAxis=[0 0 1]  RotationSequenceAxes=FollowerAxes  RotationSequence=XYX  RotationSequenceAngles=[0 0 0]  RotationSequenceAnglesUnits=deg  RotationMatrix=[1 0 0; 0 1 0; 0 0 1]  Quaternion=[1 0 0 0]  TranslationMethod=None  TranslationCartesianOffset=[0 0 0]  TranslationCartesianOffsetUnits=m  TranslationStandardAxis=+Z  TranslationStandardOffset=0  TranslationStandardOffsetUnits=m  TranslationROffset=0  TranslationROffsetUnits=m  TranslationThetaOffset=0  TranslationThetaOffsetUnits=deg  TranslationZOffset=0  TranslationZOffsetUnits=m
  Transform HandR : sm_lib/Frames and Transforms/Rigid Transform  RotationMethod=AlignedAxes  FollAlignAxisA=+Z  BaseAlignAxisA=-Y  FollAlignAxisB=+X  BaseAlignAxisB=-Z  RotationStandardAxis=+Z  RotationAngle=0  RotationAngleUnits=rad  RotationArbitraryAxis=[0 0 0]  RotationSequenceAxes=FollowerAxes  RotationSequence=XYX  RotationSequenceAngles=[0 0 0]  RotationSequenceAnglesUnits=deg  RotationMatrix=[1 0 0; 0 1 0; 0 0 1]  Quaternion=[1 0 0 0]  TranslationMethod=Cartesian  TranslationCartesianOffset=[-20 -130 -10]  TranslationCartesianOffsetUnits=mm  TranslationStandardAxis=+Z  TranslationStandardOffset=0  TranslationStandardOffsetUnits=mm  TranslationROffset=0  TranslationROffsetUnits=m  TranslationThetaOffset=0  TranslationThetaOffsetUnits=deg  TranslationZOffset=0  TranslationZOffsetUnits=m
  Transform HandR Pitch : sm_lib/Frames and Transforms/Rigid Transform  RotationMethod=StandardAxis  FollAlignAxisA=+X  BaseAlignAxisA=+Y  FollAlignAxisB=+Y  BaseAlignAxisB=+Z  RotationStandardAxis=+Z  RotationAngle=20  RotationAngleUnits=deg  RotationArbitraryAxis=[0 0 1]  RotationSequenceAxes=FollowerAxes  RotationSequence=XYX  RotationSequenceAngles=[0 0 0]  RotationSequenceAnglesUnits=deg  RotationMatrix=[1 0 0; 0 1 0; 0 0 1]  Quaternion=[1 0 0 0]  TranslationMethod=None  TranslationCartesianOffset=[0 0 0]  TranslationCartesianOffsetUnits=m  TranslationStandardAxis=+Z  TranslationStandardOffset=0  TranslationStandardOffsetUnits=m  TranslationROffset=0  TranslationROffsetUnits=m  TranslationThetaOffset=0  TranslationThetaOffsetUnits=deg  TranslationZOffset=0  TranslationZOffsetUnits=m
  Transform Steer Axis : Subsystem
  "SteerAxis  " : PMIOPort  Side=Left
  HandR : PMIOPort  Port=2  Side=Right
  HandL : PMIOPort  Port=3  Side=Right
  connections:
  Transform HandR Pitch/RConn1 -- HandR/RConn1
  Transform HandL Pitch/LConn1 -- Transform HandL/RConn1
  Solid/RConn1 -- Transform Steer Axis/RConn1
  HandL/RConn1 -- Transform HandL Pitch/RConn1
  Transform HandR/RConn1 -- Transform HandR Pitch/LConn1
  Transform Steer Axis/LConn1 -- Transform HandL/LConn1 -- Transform HandR/LConn1 -- "SteerAxis  "/RConn1

== system sm_car/Vehicle/Vehicle/Chassis/SuspA1/Linkage Decoupled/Steer/Rack Wheel Indep/Wheel/Sedan ==
  Reference Frame : sm_lib/Frames and Transforms/Reference Frame
  Steering : Subsystem
  Transform Align HandL : sm_lib/Frames and Transforms/Rigid Transform  RotationMethod=None  FollAlignAxisA=+X  BaseAlignAxisA=+Y  FollAlignAxisB=+Y  BaseAlignAxisB=+Z  RotationStandardAxis=+Z  RotationAngle=0  RotationAngleUnits=deg  RotationArbitraryAxis=[0 0 1]  RotationSequenceAxes=FollowerAxes  RotationSequence=XYX  RotationSequenceAngles=[0 0 0]  RotationSequenceAnglesUnits=deg  RotationMatrix=[1 0 0; 0 1 0; 0 0 1]  Quaternion=[1 0 0 0]  TranslationMethod=StandardAxis  TranslationCartesianOffset=[0 0 0]  TranslationCartesianOffsetUnits=m  TranslationStandardAxis=+Z  TranslationStandardOffset=0.01  TranslationStandardOffsetUnits=m  TranslationROffset=0  TranslationROffsetUnits=m  TranslationThetaOffset=0  TranslationThetaOffsetUnits=deg  TranslationZOffset=0  TranslationZOffsetUnits=m
  Transform HandL : sm_lib/Frames and Transforms/Rigid Transform  RotationMethod=ArbitraryAxis  FollAlignAxisA=+X  BaseAlignAxisA=+Y  FollAlignAxisB=+Y  BaseAlignAxisB=+Z  RotationStandardAxis=+Z  RotationAngle=0  RotationAngleUnits=rad  RotationArbitraryAxis=[0 0 0]  RotationSequenceAxes=FollowerAxes  RotationSequence=XYX  RotationSequenceAngles=[0 0 0]  RotationSequenceAnglesUnits=deg  RotationMatrix=[1 0 0; 0 1 0; 0 0 1]  Quaternion=[1 0 0 0]  TranslationMethod=Cartesian  TranslationCartesianOffset=[75.3002166748051 139.529690146446 17.4556095153098]  TranslationCartesianOffsetUnits=mm  TranslationStandardAxis=+Z  TranslationStandardOffset=0  TranslationStandardOffsetUnits=mm  TranslationROffset=0  TranslationROffsetUnits=m  TranslationThetaOffset=0  TranslationThetaOffsetUnits=deg  TranslationZOffset=0  TranslationZOffsetUnits=m
  Transform Steer Ctr : sm_lib/Frames and Transforms/Rigid Transform  RotationMethod=RotationSequence  FollAlignAxisA=+X  BaseAlignAxisA=+Y  FollAlignAxisB=+Y  BaseAlignAxisB=+Z  RotationStandardAxis=+Z  RotationAngle=0  RotationAngleUnits=deg  RotationArbitraryAxis=[0 0 1]  RotationSequenceAxes=FollowerAxes  RotationSequence=YXZ  RotationSequenceAngles=[-90 -20.218116663649042 90]  RotationSequenceAnglesUnits=deg  RotationMatrix=[1 0 0; 0 1 0; 0 0 1]  Quaternion=[1 0 0 0]  TranslationMethod=Cartesian  TranslationCartesianOffset=[0.072679731994867 0.197345148772001 0]  TranslationCartesianOffsetUnits=m  TranslationStandardAxis=+Z  TranslationStandardOffset=0  TranslationStandardOffsetUnits=m  TranslationROffset=0  TranslationROffsetUnits=m  TranslationThetaOffset=0  TranslationThetaOffsetUnits=deg  TranslationZOffset=0  TranslationZOffsetUnits=m
  Transform HandR : sm_lib/Frames and Transforms/Rigid Transform  RotationMethod=ArbitraryAxis  FollAlignAxisA=+X  BaseAlignAxisA=+Y  FollAlignAxisB=+Y  BaseAlignAxisB=+Z  RotationStandardAxis=+Z  RotationAngle=0  RotationAngleUnits=rad  RotationArbitraryAxis=[0 0 0]  RotationSequenceAxes=FollowerAxes  RotationSequence=XYX  RotationSequenceAngles=[0 0 0]  RotationSequenceAnglesUnits=deg  RotationMatrix=[1 0 0; 0 1 0; 0 0 1]  Quaternion=[1 0 0 0]  TranslationMethod=Cartesian  TranslationCartesianOffset=[75.3002166748047 139.529690146446 404.207736253739]  TranslationCartesianOffsetUnits=mm  TranslationStandardAxis=+Z  TranslationStandardOffset=0  TranslationStandardOffsetUnits=mm  TranslationROffset=0  TranslationROffsetUnits=m  TranslationThetaOffset=0  TranslationThetaOffsetUnits=deg  TranslationZOffset=0  TranslationZOffsetUnits=m
  SteerAxis : PMIOPort  Side=Left
  HandR : PMIOPort  Port=2  Side=Right
  HandL : PMIOPort  Port=3  Side=Right
  connections:
  SteerAxis/RConn1 -- Transform Steer Ctr/RConn1
  Transform HandL/RConn1 -- Transform Align HandL/LConn1
  Steering/LConn1 -- Transform Steer Ctr/LConn1
  Transform Align HandL/RConn1 -- HandL/RConn1
  Transform HandR/RConn1 -- HandR/RConn1
  Transform HandR/LConn1 -- Steering/RConn1 -- Transform HandL/LConn1
  Steering/LConn2 -- Reference Frame/RConn1
